simulink model "IMU_1"  (R2020a)
settings: Solver=FixedStepAuto  StartTime=0.0  StopTime=inf  RelTol=1e-3  EnableMultiTasking=on
libraries: arduinosensorlib x1, simulink x1
settings Model: SILPILModeSetting=veronly  ExtModeTrigDuration=2  Creator=bkhusain  LastModifiedBy=mmarathe
settings OptimizationCC: EnhancedBackFolding=on  PassReuseOutputArgsAs=Individual arguments  ZeroExternalMemoryAtStartup=off  ZeroInternalMemoryAtStartup=off  MaxStackSize=64  OptimizeBlockOrder=speed  DifferentSizesBufferReuse=on  OptimizationCustomize=off  EfficientTunableParamExpr=on
settings DebuggingCC: ParameterTunabilityLossMsg=error
settings HardwareCC: ProdBitPerPointer=32  ProdBitPerSizeT=32  ProdBitPerPtrDiffT=32  ProdLargestAtomicInteger=Long  ProdLargestAtomicFloat=Double  ProdWordSize=32  ProdHWDeviceType=ARM Compatible->ARM Cortex
settings SFSimCC: MATLABDynamicMemAlloc=off
settings RTWCC: SystemTargetFile=ert.tlc  HardwareBoard=Arduino Nano 33 IoT  TLCOptions=-aInlineSetEventsForThisBaseRateFcn=TLC_FALSE -aSuppressMultiTaskScheduler=TLC_FALSE -aRateBasedStepFcn=1  TemplateMakefile=ert_default_tmf  Toolchain=Arduino ARM  BuildConfiguration=Faster Runs
settings CodeAppCC: ForceParamTrailComments=on  IgnoreCustomStorageClasses=off  OperatorAnnotations=on  SimulinkDataObjDesc=on  SFDataObjDesc=on  InsertBlockDesc=on
settings ERTTargetCC: SupportContinuousTime=on  SupportVariableSizeSignals=on  ExtModeStaticAllocSize=8192

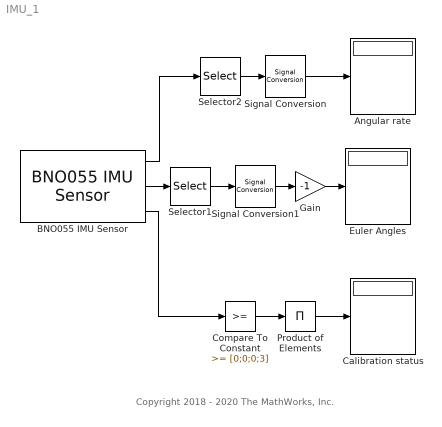
== system IMU_1 ==
  note: Copyright 2018 - 2020 The MathWorks, Inc.
  Angular rate : Display
  BNO055 IMU Sensor : arduinosensorlib/BNO055 IMU Sensor  SlaveAddress=0x28  OperationMode=Fusion  Accel=off  AngularRate=on  MagField=off  EulerAngles=on  Quat=off  LinearAccel=off  GravityVector=off  AccelRange=4G  AccelBW=62.5 Hz  GyroRange=2000 dps  GyroBW=32 Hz  MagODR=10 Hz  SampleTime=0.01  blockPlatform=ARDUINO
      settings: SourceProductBaseCode=ARDUINO
  Calibration status : Display
  Compare To Constant : simulink/Logic and Bit Operations/Compare To Constant  relop=>=  const=[0;0;0;3]  OutDataTypeStr=boolean
  Euler Angles : Display
  Gain : Gain  Gain=-1
  Product of Elements : Product  Inputs=*
  Selector1 : Selector  InputPortWidth=3  IndexOptions=Index vector (dialog)  Indices=[2]  OutputSizes=1
  Selector2 : Selector  InputPortWidth=3  IndexOptions=Index vector (dialog)  Indices=[2]  OutputSizes=1
  Signal Conversion : SignalConversion  OverrideOpt=off
  Signal Conversion1 : SignalConversion  OverrideOpt=off
  wires:
  BNO055 IMU Sensor/1 -> Selector2/1
  BNO055 IMU Sensor/2 -> Selector1/1
  BNO055 IMU Sensor/3 -> Compare To Constant/1
  Compare To Constant/1 -> Product of Elements/1
  Product of Elements/1 -> Calibration status/1
  Selector2/1 -> Signal Conversion/1
  Selector1/1 -> Signal Conversion1/1
  Signal Conversion/1 -> Angular rate/1
  Signal Conversion1/1 -> Gain/1
  Gain/1 -> Euler Angles/1
